simulink model "T13_Sim_BPSK_4"  (R2015a)
settings: Solver=ode45  StartTime=0.0  StopTime=100000  RelTol=1e-3
libraries: commdigbbndpm3 x2, commchan3 x1, commsink2 x1, commrandsrc2 x1
settings Model: Creator=User  LastModifiedBy=User

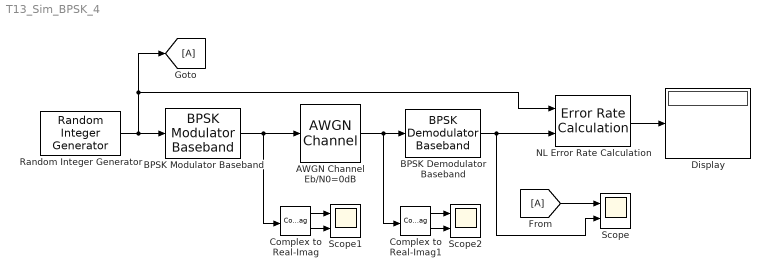
== system T13_Sim_BPSK_4 ==
  AWGN Channel Eb/N0=0dB : commchan3/AWGN Channel  InputProcessing=Columns as channels (frame based)  seed=67  noiseMode="Signal to noise ratio  (Eb/No)"  EbNodB=0  EsNodB=4  SNRdB=10  bitsPerSym=1  Ps=1  Tsym=1  variance=1
  BPSK Demodulator Baseband : commdigbbndpm3/BPSK Demodulator Baseband  Ph=0  DecType=Hard decision  VarSource=Dialog  Variance=1  outDtype=Inherit via internal rule  derotateFactorWordLen=2
  BPSK Modulator Baseband : commdigbbndpm3/BPSK Modulator Baseband  Ph=0  outDtype=double  outWordLen=16  outUDDataType=sfix(16)  outFracLenMode=Best precision  outFracLen=15
  Complex to Real-Imag : ComplexToRealImag
  Complex to Real-Imag1 : ComplexToRealImag
  Display : Display
  NL Error Rate Calculation : commsink2/Error Rate Calculation  N=0  st_delay=0  cp_mode=Entire frame  subframe=[]  PMode=Port  WsName=ErrorVec  RsMode2=off  stop=off  numErr=100  maxBits=1e6
  Random Integer Generator : commrandsrc2/Random Integer Generator  mul=2  seed=37  Ts=1  frameBased=off  sampPerFrame=1000  orient=off  outDataType=double
  Scope : Scope  NumInputPorts=2
      settings: YMin=-0.125~-0.125  YMax=1.125~1.125
  Scope1 : Scope  NumInputPorts=2
      settings: YMin=-1.25  YMax=1.25
  Scope2 : Scope  NumInputPorts=2
      settings: YMin=-3.58959  YMax=2.94404  SaveName=ScopeData2
  wires:
  Random Integer Generator/1 -> NL Error Rate Calculation/1, [A], BPSK Modulator Baseband/1
  BPSK Modulator Baseband/1 -> Complex to Real-Imag/1, AWGN Channel Eb/N0=0dB/1
  AWGN Channel Eb/N0=0dB/1 -> BPSK Demodulator Baseband/1, Complex to Real-Imag1/1
  BPSK Demodulator Baseband/1 -> NL Error Rate Calculation/2, Scope/2
  Complex to Real-Imag/1 -> Scope1/1
  Complex to Real-Imag/2 -> Scope1/2
  Complex to Real-Imag1/1 -> Scope2/1
  Complex to Real-Imag1/2 -> Scope2/2
  NL Error Rate Calculation/1 -> Display/1
  [A] -> Scope/1
